simulink model "PinCode"  (Simulink 7.7)
settings: Solver=FixedStepDiscrete  SolverMode=SingleTasking  StartTime=0.0  StopTime=10.0  FixedStep=0.001  RelTol=1e-3
libraries: dsPICdrivers x4
settings Model: Creator=ij8977  LastModifiedBy=ij8977
settings OptimizationCC: OptimizeModelRefInitCode=on  LifeSpan=1
settings RTWCC: SystemTargetFile=pic32.tlc  MakeCommand=make_CreateMPLAB  TemplateMakefile=pic32_gcc.tmf  PostCodeGenCommand=dsPIC_Compile()  Description=Embedded Target for Microchip dsPIC (real-time)  ProcessScript=pic32_make_rtw_hook
settings CodeAppCC: IgnoreCustomStorageClasses=off
settings STFCustomTargetCC: FunctionExecutionProfile=off  IncludeMdlTerminateFcn=off  CombineOutputUpdateFcns=on  SuppressErrorStatus=on  ERTCustomFileBanners=on  SupportContinuousTime=off  SupportNonInlinedSFcns=off  SystemTargetFile=pic32.tlc
settings ERTTargetCC: FunctionExecutionProfile=off  MultiwordLength=2048  ParMdlRefBuildCompliant=off  CompOptLevelCompliant=off  IncludeMdlTerminateFcn=off  SuppressErrorStatus=on  ERTFirstTimeCompliant=off  ModelStepFunctionPrototypeControlCompliant=off  CPPClassGenCompliant=off  InlinedParameterPlacement=NonHierarchical  ERTSrcFileBannerTemplate=dsPIC_code_template.cgt  ERTHdrFileBannerTemplate=dsPIC_code_template.cgt  ERTDataSrcFileTemplate=dsPIC_code_template.cgt  ERTDataHdrFileTemplate=dsPIC_code_template.cgt  ERTCustomFileTemplate=dsPIC_main.tlc  ConvertIfToSwitch=off
settings CustomProperty: DataType=string  Value=C:\PROGRA~1\MATLAB\R2011a\bin\win32\gmake

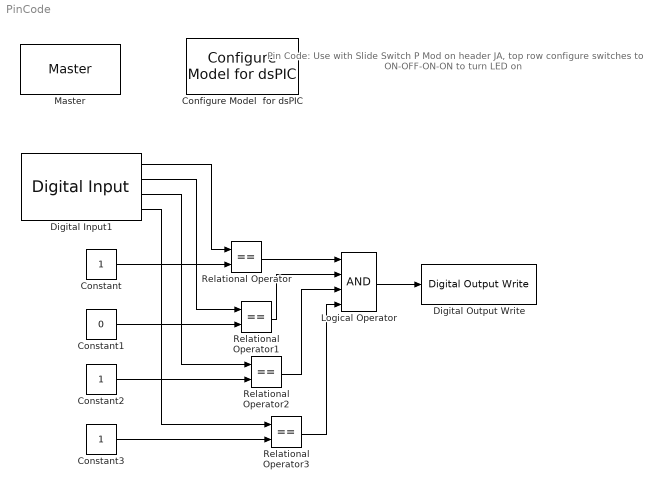
== system PinCode ==
  note: Pin Code:
      | Use with Slide Switch P Mod on header JA, top row
      | configure switches to ON-OFF-ON-ON
      | to turn LED on
  Configure Model  for dsPIC : dsPICdrivers/Simulink Configuration/Configure Model  for dsPIC
  Constant : Constant
  Constant1 : Constant  Value=0
  Constant2 : Constant
  Constant3 : Constant
  Digital Input1 : dsPICdrivers/Digital I//O/Digital Input  Tag=dsPIC_Digital_Input  PORT=E  Pin=[0; 1; 2; 3]  SampleTime=-1  OrderingInOutPopup=None
  Digital Output Write : dsPICdrivers/Digital I//O/Digital Output Write  Tag=dsPIC_Digital_Output  Priority=5  PORT=B  Pin=[10]  Simultaneous=off  OrderingInOutPopup=None
  Logical Operator : Logic  Inputs=4  AllPortsSameDT=off  OutDataTypeStr=boolean
  Master : dsPICdrivers/Master  Tag=dsPIC_MASTER  Priority=1  TimeStepType=Timer1  picType=32MX460F512L  fcy=10000000  Quartz_33f=8e6  PLLActive_33f=on  fcyDesired_33f=10e6  tmr1="[1  233  0.16]"  tmr1Info="Time Step : 0.001  ;   Error : 0%  PR1=9999"  tmr2345="[0  0  0  0]"  tmr2345cfg=[-1 -1 -1 -1]  IOautoConf=on  typePort="[ 0   0   0   0   0   0   0   0   0   0   0   0   0   0   0   0   0   0   0   0   0   0   0   0   0   0  10   0   0   0   0   0   0   0   0   0   0   0   0   0   0   0   0   0   0   0   0   0   0   0   0   0   0   0   0   0   0   0   0   0   0   0   0   0   9   9   9   9   0   0   0   0   0   0   0   0   0   0   0   0   0   0   0   0   0   0   0   0   0   0   0   0   0   0   0   0   0   0   0   0   0   0   0   0   0   0   0   0   0   0   0   0 ]"  TRIS="[ 65535  64511  65535  65535  65535  65535  65535 ]"  ADPCFG=1024  MasterBusyPort=None  MasterOverloadPort=None  FOSC=Quartz (XT - HS)  ClockSwitchMonitor=Both disabled  TempProtection_33f=TEMP_ON  FPBOR=<empty>  PWRT=disable  MCLR=<empty>  ICD=ICS_PGD1  JTAGEN=JTAGEN_OFF  PowerSave=off  OverrideFcy=off  NewFcy=1e6  PR2345="[65535  65535  65535  65535]"
  Relational Operator{,1..3} (4 alike) : RelationalOperator  Operator===  OutDataTypeStr=boolean
  wires:
  Relational Operator/1 -> Logical Operator/1
  Digital Input1/1 -> Relational Operator/1
  Constant/1 -> Relational Operator/2
  Digital Input1/2 -> Relational Operator1/1
  Digital Input1/3 -> Relational Operator2/1
  Digital Input1/4 -> Relational Operator3/1
  Constant1/1 -> Relational Operator1/2
  Constant2/1 -> Relational Operator2/2
  Constant3/1 -> Relational Operator3/2
  Relational Operator1/1 -> Logical Operator/2
  Relational Operator2/1 -> Logical Operator/3
  Relational Operator3/1 -> Logical Operator/4
  Logical Operator/1 -> Digital Output Write/1
